simulink model "Position_controller_enable_disable"  (Simulink 8.1)
settings: Solver=ode4  SolverMode=SingleTasking  StartTime=0.0  StopTime=inf  FixedStep=BKIN_STEP_TIME  RelTol=1e-3
model workspace (MAT data in the model file):
  BKIN_STEP_TIME = 0.0005
  col_x = 1
  col_y = 2
  VRAD = 3
  COLOR = 4
  TARGET_COL = 2
  TRAJ_DURATION_COL = 3
  POSITION_RAMP_TIME = 1
  START_TARGET = 1
  WAIT_FOR_ENABLE = 5
  ENABLED_CONTROLLER = 6
  MOVING = 7
  DONE_MOVEMENT = 8
  WAIT_AT_START_TIME : num (value not decoded)
StartFcn:
  |  warndlg('Dexterit-E models cannot run under simulation. Please compile your model and run it from within Dexterit-E.');set_param(bdroot,'SimulationCommand','stop')
libraries: General x3, Video x3, simulink x3, KINARM_general x2, KINARM_EP_loads x2, KINARM_loads x1
CloseFcn:
  | rtwprivate ssgencode ModelCloseRequest b2lab2d
settings Model: Creator=Chris Grebeldinger  LastModifiedBy=BKIN TECHNOLOGIES  ModifiedComment=chris -- Wed Feb 16 09:18:30 2005 -- Version 1.1384  ModifiedHistory=Feb 16/05 - Add error repeat, add offset ramp  ExtModeArmWhenConnect=off  ExtModeLogAll=off  BufferReuse=off
settings SolverCC: AutoInsertRateTranBlk=on
settings DataIOCC: LimitDataPoints=off  SaveOutput=off  SaveTime=off  SignalLoggingName=sigsOut
settings OptimizationCC: BlockReduction=off  BooleanDataType=off  OptimizeBlockIOStorage=off  BufferReuse=off  ExpressionFolding=off  FoldNonRolledExpr=off  LocalBlockOutputs=off  InitFltsAndDblsToZero=on
settings DebuggingCC: SaveWithParameterizedLinksMsg=none  SignalResolutionControl=TryResolveAllWithWarning  SolverPrmCheckMsg=none  MultiTaskDSMMsg=warning  MultiTaskCondExecSysMsg=none  StrictBusMsg=None
settings HardwareCC: ProdIntDivRoundTo=Zero  ProdEndianess=LittleEndian  ProdHWDeviceType=Generic->32-bit x86 compatible  TargetHWDeviceType=32-bit Generic
settings SFSimCC: SimParseCustomCode=off
settings RTWCC: SystemTargetFile=xpctarget.tlc  TemplateMakefile=xpc_default_tmf  Description=xPC Target  ProcessScript=xpctarget_make_rtw_hook  IncludeERTFirstTime=on  RTWCompilerOptimization=On
settings CodeAppCC: MaxIdLength=63
settings xpcTargetCC: TargetFcnLib=ansi_tfl_tmw.mat  CodeReplacementLibrary=XPC_BLAS  ParMdlRefBuildCompliant=on  ConcurrentExecutionCompliant=on  CombineSignalStateStructs=off  MATLABClassNameForMDSCustomization=xpcAperiodicCustomization  GRTInterface=on  GenerateAllocFcn=off  xPCTaskExecutionProfile=off  xPCRL32EventNumber=5000  xPCisDownloadable=off  xPCLoadParamSetFile=off  xPCConcurrentTasks=off  xPCEnableSFAnimation=off

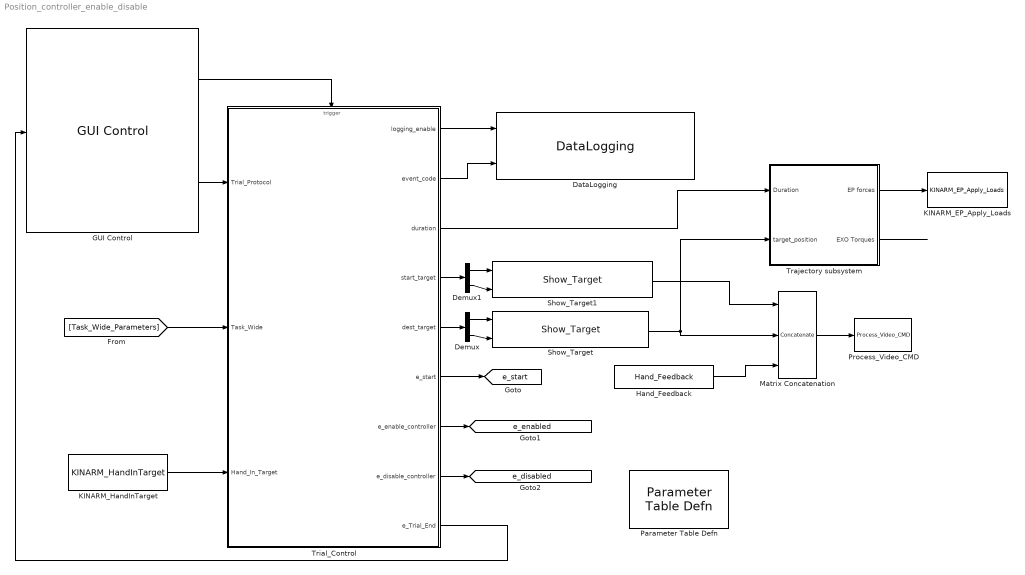
== system Position_controller_enable_disable ==
  DataLogging : General/DataLogging  log_event_codes=on  log_analog_inputs=off
      link override Poll KINARM/EPTorqueCMD: GotoTag=KINARMEPTorqueCMD
  Demux : Demux  Outputs=2
  Demux1 : Demux  Outputs=2
  GUI Control : General/GUI Control  target_type_str=Circle  Target_Type=1  XYcols=[1 2]  Vcols=3  Lcols=4  indices_padding=[0 0 0 0;0 0 0 0]  task_version=1.0  show_repeat_trial_flag=off
  Hand_Feedback : KINARM_general/Hand_Feedback  feedback_cntl_src=none
  KINARM_EP_Apply_Loads : KINARM_EP_loads/KINARM_EP_Apply_Loads  up_duration=1500  down_duration=1500  max_force=60
  KINARM_HandInTarget : KINARM_general/KINARM_HandInTarget  use_dominant_hand=on  target_type=Circle  num_states=1  attribcol1=[VRAD]  attribcol2=[3]  attribcol3=[3]  attribcol4=[3]  attribcol5=[0]
  Matrix Concatenation : Concatenate  NumInputs=3  Mode=Multidimensional array
  Parameter Table Defn : General/Parameter Table Defn  ShowInLibBrowser=0
  Process_Video_CMD : Video/Process_Video_CMD
  Show_Target : Video/Show_Target  target_type=Circle  num_states=1  attribcol1=[COLOR 0 0 VRAD]  attribcol2=[5 0 0 3]  attribcol3=[0 0 0 0]  attribcol4=[0 0 0 0]  attribcol5=[0 0 24 0]  stateindices_padding=[0 0 0 0 0 0 0;0 0 0 0 0 0 0;0 0 0 0 0 0 0;0 0 0 0 0 0 0;0 0 0 0 0 0 0]  source=dialog  opacity=100  target_display=Both subject and operator displays  num_col=4
  Show_Target1 : Video/Show_Target  target_type=Circle  num_states=1  attribcol1=[COLOR 0 0 VRAD]  attribcol2=[5 0 0 3]  attribcol3=[0 0 0 0]  attribcol4=[0 0 0 0]  attribcol5=[0 0 24 0]  stateindices_padding=[0 0 0 0 0 0 0;0 0 0 0 0 0 0;0 0 0 0 0 0 0;0 0 0 0 0 0 0;0 0 0 0 0 0 0]  source=dialog  opacity=100  target_display=Both subject and operator displays  num_col=4
  Trajectory subsystem : Subsystem
  Trial_Control : Stateflow chart  TreatAsAtomicUnit=on
  tag scope: e_disabled=global, e_enabled=global, e_start=global
  wires:
  Show_Target/1 -> Matrix Concatenation/2, Trajectory subsystem/2(target_position)
  Trial_Control/9(e_Trial_End) -> GUI Control/1
  GUI Control/1 -> Trial_Control/Trigger
  Matrix Concatenation/1 -> Process_Video_CMD/1
  GUI Control/2 -> Trial_Control/1(Trial_Protocol)
  Trial_Control/1(logging_enable) -> DataLogging/1
  Trial_Control/3(duration) -> Trajectory subsystem/1(Duration)
  Trajectory subsystem/1(EP forces) -> KINARM_EP_Apply_Loads/1
  Trajectory subsystem/2(EXO Torques) -> ?
  Trial_Control/6(e_start) -> [e_start]
  Trial_Control/7(e_enable_controller) -> [e_enabled]
  Trial_Control/8(e_disable_controller) -> [e_disabled]
  [Task_Wide_Parameters] -> Trial_Control/2(Task_Wide)
  KINARM_HandInTarget/1 -> Trial_Control/3(Hand_In_Target)
  Demux/1 -> Show_Target/1
  Demux/2 -> Show_Target/2
  Trial_Control/5(dest_target) -> Demux/1
  Demux1/1 -> Show_Target1/1
  Trial_Control/4(start_target) -> Demux1/1
  Demux1/2 -> Show_Target1/2
  Trial_Control/2(event_code) -> DataLogging/2
  Show_Target1/1 -> Matrix Concatenation/1
  Hand_Feedback/1 -> Matrix Concatenation/3

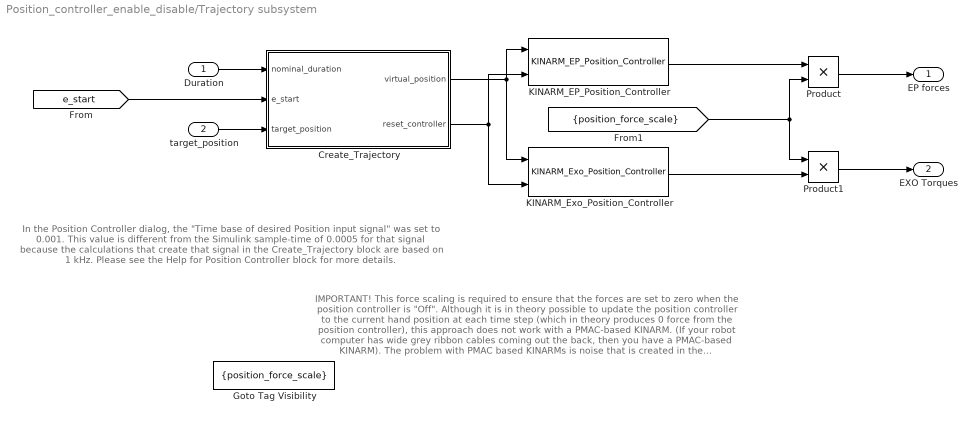
== system Position_controller_enable_disable/Trajectory subsystem ==
  note: IMPORTANT! This force scaling is required to ensure that the forces are set to zero when the position controller is "Off".
      | Although it is in theory possible to update the position controller to the current hand position at each time step (which
      | in theory produces 0 force from the position controller), this approach does not work with a PMAC-based KINARM.
      | (If your robot computer has wide grey ribbon cables coming out the back, then you have a PMAC-based KINARM).
      | The problem with PMAC based KINARMs is noise that is created in the virtual_postion, which is caused by the PMAC sampling
      | at 1129 Hz and the model running at 2 kHz (i.e. data are re-sampled). These differences mean that time base used by the
      | position controller to calculate velocity is incorrect. It should be 884 us, but instead is 500 us. As such, at 2nd or third frame you
      | can see the position may hold. This re-sampling leads to high instantaneous velocities intermingled with v = 0. There is no way
      | around this on a PMAC system. Therefore you need to disable the position controller's forces if you want the subject to move freely
  note: In the Position Controller dialog, the "Time base of desired Position input signal" was set to 0.001.
      | This value is different from the Simulink sample-time of 0.0005 for that signal because the calculations
      | that create that signal in the Create_Trajectory block are based on 1 kHz. Please see the Help for
      | Position Controller block for more details.
  Duration : Inport
  target_position : Inport  Port=2
  Create_Trajectory : Subsystem
  Goto Tag Visibility : GotoTagVisibility  GotoTag=position_force_scale
  KINARM_EP_Position_Controller : KINARM_EP_loads/KINARM_EP_Position_Controller  use_dom_hand=on  inertias_for_FF=KINARM End Point robot  gain_choice=Standard Movement  sample_time=0.001
  KINARM_Exo_Position_Controller : KINARM_loads/KINARM_Exo_Position_Controller  use_dom_hand=on  KINARM_Type=Human  inertias_for_FF=KINARM robot  angles_or_XY=End-point (global x/y)  sample_time=0.001
  Product : Product
  Product1 : Product
  EP forces : Outport
  EXO Torques : Outport  Port=2
  wires:
  Create_Trajectory/2(reset_controller) -> KINARM_Exo_Position_Controller/2, KINARM_EP_Position_Controller/2
  Create_Trajectory/1(virtual_position) -> KINARM_EP_Position_Controller/1, KINARM_Exo_Position_Controller/1
  KINARM_EP_Position_Controller/1 -> Product/1
  KINARM_Exo_Position_Controller/1 -> Product1/2
  target_position/1 -> Create_Trajectory/3(target_position)
  Duration/1 -> Create_Trajectory/1(nominal_duration)
  [e_start] -> Create_Trajectory/2(e_start)
  Product/1 -> EP forces/1
  Product1/1 -> EXO Torques/1
  [position_force_scale] -> Product1/1, Product/2

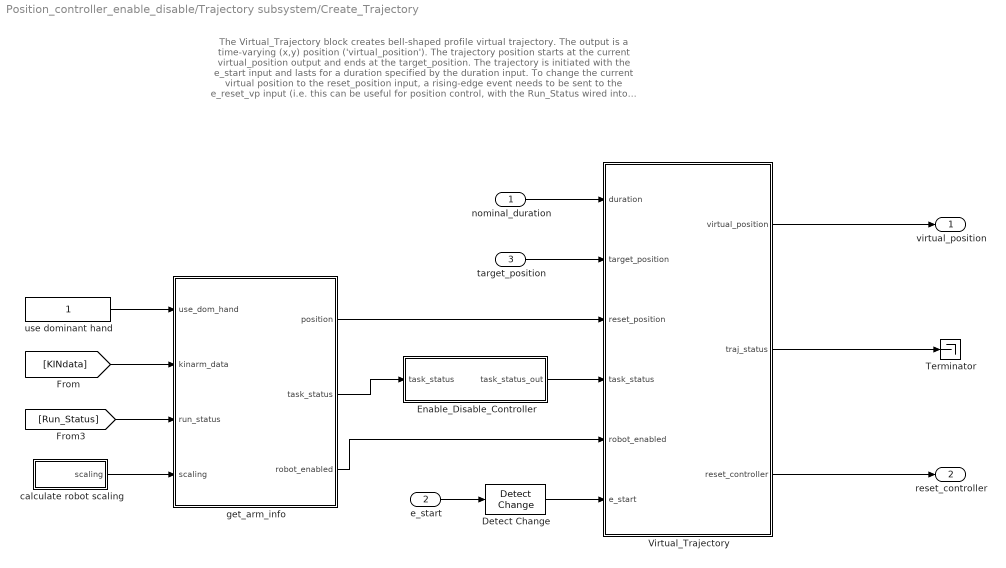
== system Position_controller_enable_disable/Trajectory subsystem/Create_Trajectory ==
  note: The Virtual_Trajectory block creates bell-shaped profile virtual trajectory.
      | The output is a time-varying (x,y) position ('virtual_position').
      |
      | The trajectory position starts at the current virtual_position output and ends at the target_position.
      | The trajectory is initiated with the e_start input and lasts for a duration specified by the duration input.
      |
      | To change the current virtual position to the reset_position input, a rising-edge event needs to be sent to the e_reset_vp input
      | (i.e. this can be useful for position control, with the Run_Status wired into the e_reset input).
      | If such an event occurs during a virtual trajectory, the trajectory is halted immediately.
  nominal_duration : Inport
  e_start : Inport  Port=2
  target_position : Inport  Port=3
  Detect Change : simulink/Logic and Bit Operations/Detect Change  vinit=0  InputProcessing=Inherited  OutDataTypeStr=uint8
  Enable_Disable_Controller : Subsystem
  Terminator : Terminator
  Virtual_Trajectory : Subsystem
  calculate robot scaling : Subsystem
  get_arm_info : MATLAB Function  TreatAsAtomicUnit=on
  use dominant hand : Constant
  virtual_position : Outport
  reset_controller : Outport  Port=2
  wires:
  nominal_duration/1 -> Virtual_Trajectory/1(duration)
  e_start/1 -> Detect Change/1
  target_position/1 -> Virtual_Trajectory/2(target_position)
  Detect Change/1 -> Virtual_Trajectory/6(e_start)
  use dominant hand/1 -> get_arm_info/1(use_dom_hand)
  [KINdata] -> get_arm_info/2(kinarm_data)
  Virtual_Trajectory/3(reset_controller) -> reset_controller/1
  get_arm_info/2(task_status) -> Enable_Disable_Controller/1(task_status)
  get_arm_info/3(robot_enabled) -> Virtual_Trajectory/5(robot_enabled)
  [Run_Status] -> get_arm_info/3(run_status)
  Virtual_Trajectory/2(traj_status) -> Terminator/1
  calculate robot scaling/1(scaling) -> get_arm_info/4(scaling)
  Enable_Disable_Controller/1(task_status_out) -> Virtual_Trajectory/4(task_status)
  get_arm_info/1(position) -> Virtual_Trajectory/3(reset_position)
  Virtual_Trajectory/1(virtual_position) -> virtual_position/1

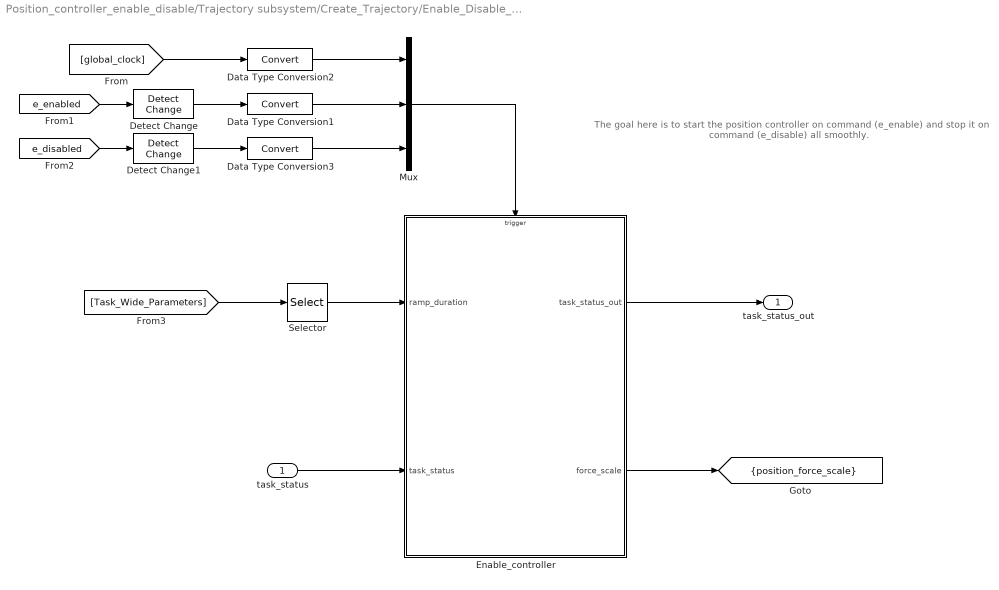
== system Position_controller_enable_disable/Trajectory subsystem/Create_Trajectory/Enable_Disable_Controller ==
  note: The goal here is to start the position controller on command (e_enable)
      | and stop it on command (e_disable) all smoothly.
  task_status : Inport
  Data Type Conversion1 : DataTypeConversion
  Data Type Conversion2 : DataTypeConversion
  Data Type Conversion3 : DataTypeConversion
  Detect Change : simulink/Logic and Bit Operations/Detect Change  vinit=0  InputProcessing=Inherited  OutDataTypeStr=uint8
  Detect Change1 : simulink/Logic and Bit Operations/Detect Change  vinit=0  InputProcessing=Inherited  OutDataTypeStr=uint8
  Enable_controller : Stateflow chart  TreatAsAtomicUnit=on
  Mux : Mux  Inputs=3
  Selector : Selector  IndexOptions=Index vector (dialog)  Indices=[POSITION_RAMP_TIME]  OutputSizes=1
  task_status_out : Outport
  tag scope: position_force_scale=scoped
  wires:
  [e_enabled] -> Detect Change/1
  [global_clock] -> Data Type Conversion2/1
  Mux/1 -> Enable_controller/Trigger
  Selector/1 -> Enable_controller/1(ramp_duration)
  Data Type Conversion2/1 -> Mux/1
  task_status/1 -> Enable_controller/2(task_status)
  Data Type Conversion1/1 -> Mux/2
  [e_disabled] -> Detect Change1/1
  Data Type Conversion3/1 -> Mux/3
  Enable_controller/2(force_scale) -> [position_force_scale]
  Enable_controller/1(task_status_out) -> task_status_out/1
  Detect Change/1 -> Data Type Conversion1/1
  Detect Change1/1 -> Data Type Conversion3/1
  [Task_Wide_Parameters] -> Selector/1

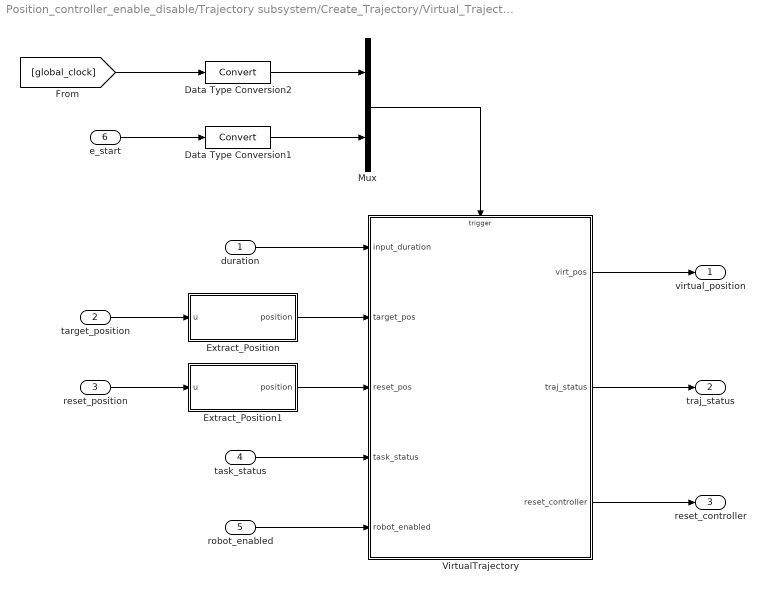
== system Position_controller_enable_disable/Trajectory subsystem/Create_Trajectory/Virtual_Trajectory ==
  duration : Inport
  target_position : Inport  Port=2
  reset_position : Inport  Port=3
  task_status : Inport  Port=4
  robot_enabled : Inport  Port=5
  e_start : Inport  Port=6
  Data Type Conversion1 : DataTypeConversion
  Data Type Conversion2 : DataTypeConversion
  Extract_Position : MATLAB Function  TreatAsAtomicUnit=on
  Extract_Position1 : MATLAB Function  TreatAsAtomicUnit=on
  Mux : Mux  Inputs=2
  VirtualTrajectory : Stateflow chart  TreatAsAtomicUnit=on
  virtual_position : Outport
  traj_status : Outport  Port=2
  reset_controller : Outport  Port=3
  wires:
  e_start/1 -> Data Type Conversion1/1
  target_position/1 -> Extract_Position/1(u)
  [global_clock] -> Data Type Conversion2/1
  Mux/1 -> VirtualTrajectory/Trigger
  duration/1 -> VirtualTrajectory/1(input_duration)
  VirtualTrajectory/1(virt_pos) -> virtual_position/1
  Extract_Position/1(position) -> VirtualTrajectory/2(target_pos)
  reset_position/1 -> Extract_Position1/1(u)
  Data Type Conversion2/1 -> Mux/1
  VirtualTrajectory/2(traj_status) -> traj_status/1
  robot_enabled/1 -> VirtualTrajectory/5(robot_enabled)
  task_status/1 -> VirtualTrajectory/4(task_status)
  Data Type Conversion1/1 -> Mux/2
  Extract_Position1/1(position) -> VirtualTrajectory/3(reset_pos)
  VirtualTrajectory/3(reset_controller) -> reset_controller/1

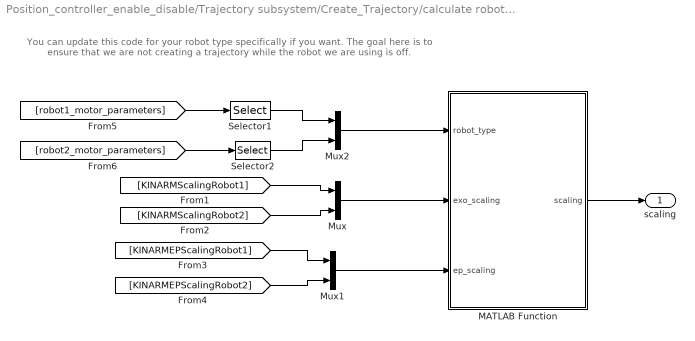
== system Position_controller_enable_disable/Trajectory subsystem/Create_Trajectory/calculate robot scaling ==
  note: You can update this code for your robot type specifically if you want. The goal here
      | is to ensure that we are not creating a trajectory  while the robot we are using is off.
  MATLAB Function : MATLAB Function  TreatAsAtomicUnit=on
  Mux : Mux  Inputs=2
  Mux1 : Mux  Inputs=2
  Mux2 : Mux  Inputs=2
  Selector1 : Selector  InputPortWidth=9  IndexOptions=Index vector (dialog)  Indices=[7]  OutputSizes=[(-2)]
  Selector2 : Selector  InputPortWidth=9  IndexOptions=Index vector (dialog)  Indices=[7]  OutputSizes=[(-2)]
  scaling : Outport
  wires:
  [KINARMScalingRobot1] -> Mux/1
  [KINARMScalingRobot2] -> Mux/2
  Mux/1 -> MATLAB Function/2(exo_scaling)
  Mux1/1 -> MATLAB Function/3(ep_scaling)
  Mux2/1 -> MATLAB Function/1(robot_type)
  MATLAB Function/1(scaling) -> scaling/1
  [robot2_motor_parameters] -> Selector2/1
  [KINARMEPScalingRobot2] -> Mux1/2
  [KINARMEPScalingRobot1] -> Mux1/1
  [robot1_motor_parameters] -> Selector1/1
  Selector1/1 -> Mux2/1
  Selector2/1 -> Mux2/2

== stateflow chart Trial_Control ==
  settings: sampleTime=0.001
  state EndOfTrial/
    //ramp the position controller off slowly now
    e_disable_controller;
  state init/
    logging_enable = 1;
    controller_on = 0;
  state Inter_Trial_State/
    e_Trial_End
    start_target[2] = 0;
    dest_target[2] = 0;
    controller_on = 0;
  state Main_Trial
    state MoveLoadedArm/
      e_start;
      event_code = MOVING;
    state ShowDestination/
      dest_target[1] = Trial_Protocol[TARGET_COL];
      dest_target[2] = 1;
      duration =Trial_Protocol[TRAJ_DURATION_COL];
    state WaitForStart/
      start_target[1] = Trial_Protocol[START_TARGET];
      start_target[2] = 1; //show the start target
      event_code = WAIT_FOR_ENABLE;
      ramp_time = Task_Wide[POSITION_RAMP_TIME];
      wait_at_target = Task_Wide[WAIT_AT_START_TIME];
    state EnableController/
      //Stop the subject in their current location so the trajectory can start from there
      //then allow the position controller to ramp on slowly
      e_enable_controller;
      start_target[2] = 0; //hide the start target
      event_code = ENABLED_CONTROLLER;
      controller_on = 1;
    state StopAtTarget/
      //Wait for the subject to stabilize in the start target
      //This makes turning on the controller feel better
    state WaitAtTarget/
      event_code = DONE_MOVEMENT;
    WaitForStart -> StopAtTarget : [Hand_In_Target[start_target[1]] == 1]
    StopAtTarget -> WaitForStart [order 2] : [Hand_In_Target[start_target[1]] != 1]
    StopAtTarget -> EnableController [order 1] : after(wait_at_target, e_clk)
    EnableController -> ShowDestination : after(ramp_time + wait_at_target, e_clk)
    ShowDestination -> MoveLoadedArm : after(2, e_clk)
    MoveLoadedArm -> WaitAtTarget : after(duration, e_clk)
  (default) -> init
  init -> WaitForStart
  Inter_Trial_State -> WaitForStart
  (junction 36) -> Inter_Trial_State [order 2]
  EndOfTrial -> Inter_Trial_State : after(ramp_time, e_clk)
  Main_Trial -> (junction 36) : e_ExitTrialNow
  (junction 36) -> EndOfTrial [order 1] : [controller_on == 1]
  WaitAtTarget -> EndOfTrial : after(wait_at_target, e_clk)
  data: logging_enable output boolean; event_code output double; duration output double; start_target output double size=[1 2] =zeros(1, 2); dest_target output double size=[1 2] [1..32] =zeros(1, 2); ramp_time local double; Trial_Protocol input double; Task_Wide input double; Hand_In_Target input double; wait_at_target local double; controller_on local double
  data dest_target settings: description=index of the row currently being used in the TargetTable
  events: e_start output EITHER_EDGE_EVENT; e_clk input RISING_EDGE_EVENT; e_ExitTrialNow input EITHER_EDGE_EVENT; e_enable_controller output EITHER_EDGE_EVENT; e_disable_controller output EITHER_EDGE_EVENT; e_Trial_End output EITHER_EDGE_EVENT

== matlab function Trajectory subsystem/Create_Trajectory/calculate robot scaling/MATLAB Function ==
  data: robot_type input double; scaling output double; exo_scaling input double; ep_scaling input double
function scaling = fcn(robot_type, exo_scaling, ep_scaling)
%#codegen

scaling = [0, 0];

%0 = EXO, 1 = EP, 2 = NHP
for n=1:2
    if robot_type(n) == 1
        scaling(n) = ep_scaling(n);
    else
        scaling(n) = exo_scaling(n);
    end
end

== matlab function Trajectory subsystem/Create_Trajectory/Virtual_Trajectory/Extract_Position ==
  settings: fimath=|
      | fimath(...
      | 'RoundMode', 'floor',...
      | 'OverflowMode', 'wrap',...
      | 'ProductMode', 'KeepLSB', 'ProductWordLength', 32,...
      | 'SumMode', 'KeepLSB', 'SumWordLength', 32,...
      | 'CastBeforeSum', false)
  data: u input double; position output double
function position = fcn(u)

position=[0,0];	%initialization
if length(u)==2	%input is assumed to be (x,y) position, global coordinates, (m)		
	position=u;
else			%input is assumed to be a VCODE
	position(1)=u(3);
	position(2)=u(4);
end

== matlab function Trajectory subsystem/Create_Trajectory/Virtual_Trajectory/Extract_Position1 ==
  settings: fimath=|
      | fimath(...
      | 'RoundMode', 'floor',...
      | 'OverflowMode', 'wrap',...
      | 'ProductMode', 'KeepLSB', 'ProductWordLength', 32,...
      | 'SumMode', 'KeepLSB', 'SumWordLength', 32,...
      | 'CastBeforeSum', false)
  data: u input double; position output double
function position = fcn(u)

position=[0,0];	%initialization
if length(u)==2	%input is assumed to be (x,y) position, global coordinates, (m)		
	position=u;
else			%input is assumed to be a VCODE
	position(1)=u(3);
	position(2)=u(4);
end

== stateflow chart Trajectory subsystem/Create_Trajectory/Virtual_Trajectory/VirtualTrajectory ==
  state main/
    state wait_for_trigger/
      reset_controller = 0;
      traj_status = 1;
    state on_ramp/
      entry: tick = 0;    // initialize the tick counter
      reset_controller = 0;
      final_pos = target_pos;   // set the final position of the trajectory
      start_pos = virt_pos;   // set the start position of the trajectory
      duration = input_duration;   // store the duration of the trajectory
      traj_status = 3;   // indicate an ongoing trajectory
      during:
      on e_clk: tick++;
      // the trajectory velocity will have a bell shaped profile
      trajectory_shape = tick/duration-sin(2*pi*tick/duration)/(2*pi);
      virt_pos[1] = start_pos[1] + (final_pos[1] - start_pos[1]) * trajectory_shape;
      virt_pos[2] = start_pos[2] + (final_pos[2] - start_pos[2]) * trajectory_shape;
    state wait_1_ms_b/
      // wait for controller
      // to be reset
      traj_status = 2;
    main -> wait_1_ms_b [order 1] : [(robot_enabled == 1) && (traj_status == -1)]/
        | traj_status = 1;
        | virt_pos = reset_pos;
        | reset_controller = 1;
        | // trajectory was halted and
        | //is now being re-started
    wait_for_trigger -> (junction 77) : e_start
    (junction 77) -> wait_for_trigger [order 2]
    wait_1_ms_b -> (junction 77) : after(1, e_clk)
    (junction 77) -> on_ramp [order 1] : [input_duration>0]
    on_ramp -> wait_for_trigger [order 2] : [robot_enabled == 0]/
        | traj_status = -1;
        | // robot disabled
    on_ramp -> wait_for_trigger [order 1] : after(duration, e_clk)/
        | traj_status = 0
        | // trajectory completed
  state Initialization/
    virt_pos = reset_pos;
    // this initialization ensures that the virtual position
    // starts off as something reasonable
    traj_status = 0;   // initialize trajectory status
  state task_not_running/
    // wait for task_status to change
    // keep updating virt_pos so that the feedback
    // controller output, which is filtered, does not become
    // huge, resulting in a 'bump' if we don't do this.
    traj_status = 4;
    reset_controller = 0;
    during:
    virt_pos = reset_pos;
  state wait_1_ms/
    // wait for controller
    // to be reset
    traj_status = 5;
  (default) -> Initialization
  Initialization -> wait_for_trigger
  wait_1_ms -> wait_for_trigger : after(1, e_clk)
  task_not_running -> wait_1_ms : [task_status > 0]/
      | reset_controller = 1;
      | // task is running again,
      | // so reset position controller
  main -> task_not_running [order 1] : [task_status == 0]/
      | // means that run_status == 0
      | // AND that torque scaling at
      | // end of task is finished
  data: input_duration input double; target_pos input double size=[1 2]; tick local double; duration local double; reset_pos input double size=[1 2]; task_status input double; pi constant double =3.14159265358979; trajectory_shape local double; virt_pos output double size=[1 2]; traj_status output double; robot_enabled input double; start_pos local double size=[1 2]; final_pos local double size=[1 2]; reset_controller output double
  events: e_clk input RISING_EDGE_EVENT; e_start input RISING_EDGE_EVENT

== matlab function Trajectory subsystem/Create_Trajectory/get_arm_info ==
  settings: fimath=|
      | fimath(...
      | 'RoundMode', 'floor',...
      | 'OverflowMode', 'wrap',...
      | 'ProductMode', 'KeepLSB', 'ProductWordLength', 32,...
      | 'SumMode', 'KeepLSB', 'SumWordLength', 32,...
      | 'CastBeforeSum', false)
  data: position output double; task_status output double; use_dom_hand input double; kinarm_data input double; run_status input double; scaling input double; robot_enabled output double
function [position, task_status, robot_enabled]  = fcn(use_dom_hand, kinarm_data, run_status, scaling)
%
% get current hand position and robot enabled status
%
% May 2009
%

hpx_index = 23;
hpy_index = 24;
robot_disabled_index = 37;

%determine which arm to apply the load to
dominant_hand=kinarm_data(3,1);						%kinarm_data(3,1) tells which arm is the dominant arm
if use_dom_hand == 1
	feedback_arm = dominant_hand;
else
	feedback_arm = 3 - dominant_hand;
end

hpx = kinarm_data( feedback_arm, hpx_index );
hpy = kinarm_data( feedback_arm, hpy_index );
position = [hpx hpy];

if kinarm_data( feedback_arm, robot_disabled_index ) == 0;
    robot_enabled = 1;
else
    robot_enabled = 0;
end

% if the task has stopped/paused (i.e. run_status == 0) AND the torques outputs
% have scaled down to 0, then set the task_status = 0.
if run_status == 0 && scaling(feedback_arm) == 0
    task_status = 0;
else
    task_status = 1;
end

== stateflow chart Trajectory subsystem/Create_Trajectory/Enable_Disable_Controller/Enable_controller ==
  state Initialization/
    force_scale = 0;
    task_status_out = 0;
  state Start_enable/
    ramp_amount = 1 / ramp_duration;
    during:
    on e_clk: force_scale = force_scale + ramp_amount;
  state WaitForStatus/
    task_status_out = 1;
  state WaitWhileOn/
    force_scale =1;
  state Start_Diasble/
    ramp_amount = 1 / ramp_duration;
    during:
    on e_clk: force_scale = force_scale - ramp_amount;
  (default) -> Initialization
  Start_Diasble -> Initialization : [force_scale <= 0]
  Initialization -> WaitForStatus : e_enable
  WaitForStatus -> Start_enable : [task_status == 1]
  Start_enable -> WaitWhileOn : [force_scale >= 1]
  WaitWhileOn -> Start_Diasble : e_disable
  data: ramp_duration input double; task_status input double; task_status_out output double; force_scale output double; ramp_amount local double
  events: e_clk input RISING_EDGE_EVENT; e_enable input RISING_EDGE_EVENT; e_disable input RISING_EDGE_EVENT
